simulink model "PIC_vector_concatenate_test"  (Simulink 6.6)
settings: Solver=FixedStepDiscrete  StartTime=0.0  StopTime=10.0  FixedStep=0.00001  RelTol=1e-3
libraries: dsPICdrivers x9, commutil2 x1, simulink x1
settings Model: Creator=Corey  LastModifiedBy=Corey  ProdHWDeviceType=16-bit Generic
settings OptimizationCC: OptimizeModelRefInitCode=on  LifeSpan=1
settings HardwareCC: ProdBitPerInt=16  ProdEndianess=LittleEndian  ProdWordSize=16  ProdHWDeviceType=16-bit Generic  TargetHWDeviceType=32-bit Generic
settings RTWCC: SystemTargetFile=dspic.tlc  TemplateMakefile=dspic_pic30_gcc.tmf  PostCodeGenCommand=dsPIC_Compile()  Description=Embedded Target for Microchip dsPIC (real-time)  ProcessScript=dspic_make_rtw_hook
settings CodeAppCC: IgnoreCustomStorageClasses=off
settings STFCustomTargetCC: TargetFcnLib=ansi_tfl_tmw.mat  GenFloatMathFcnCalls=ANSI_C  ModelReferenceCompliant=off  IncludeMdlTerminateFcn=off  CombineOutputUpdateFcns=on  SuppressErrorStatus=on  ERTCustomFileBanners=on  SupportContinuousTime=off  SupportNonInlinedSFcns=off  SystemTargetFile=dspic.tlc
settings ERTTargetCC: TargetFcnLib=ansi_tfl_tmw.mat  GenFloatMathFcnCalls=ANSI_C  ModelReferenceCompliant=off  IncludeMdlTerminateFcn=off  SuppressErrorStatus=on  ModelStepFunctionPrototypeControlCompliant=off  ExtModeMexFile=noextcomm  InlinedParameterPlacement=NonHierarchical  ERTSrcFileBannerTemplate=dsPIC_code_template.cgt  ERTHdrFileBannerTemplate=dsPIC_code_template.cgt  ERTDataSrcFileTemplate=dsPIC_code_template.cgt  ERTDataHdrFileTemplate=dsPIC_code_template.cgt  ERTCustomFileTemplate=dsPIC_main.tlc
settings CustomProperty: DataType=string  Value=J:\PROGRA~1\MATLAB\R2007a\rtw\bin\win32\gmake

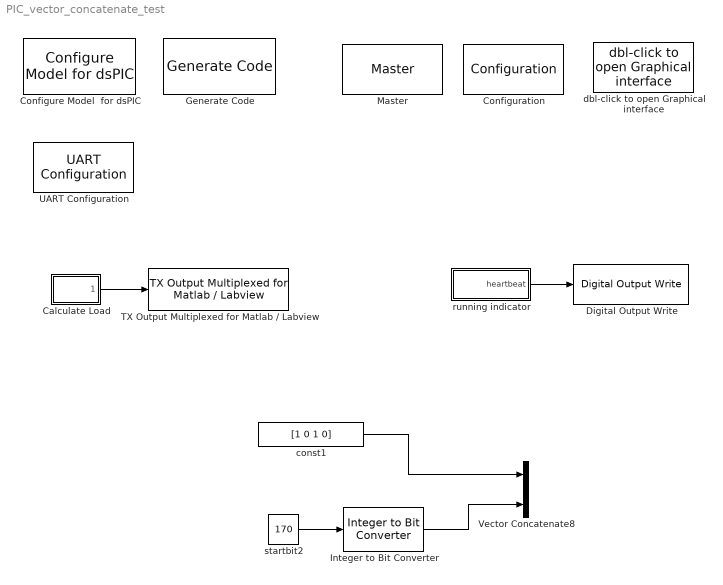
== system PIC_vector_concatenate_test ==
  Calculate Load : Subsystem
  Configuration : dsPICdrivers/Configuration  SystemSampleTime=-1  double64=off
  Configure Model  for dsPIC : dsPICdrivers/Simulink Configuration/Configure Model  for dsPIC
  Digital Output Write : dsPICdrivers/Digital I//O/Digital Output Write  Tag=dsPIC_Digital_Output  Priority=5  PORT=A  Pin=[0]  Simultaneous=off  OrderingInOutPopup=None
  Generate Code : dsPICdrivers/Simulink Configuration/Generate Code
  Integer to Bit Converter : commutil2/Integer to Bit Converter  nbits=8  outDtype=boolean
  Master : dsPICdrivers/Master  Tag=dsPIC_MASTER  Priority=1  TimeStepType=Timer1  picType=33fJ256GP710  fcy=40000000  Quartz_33f=8e6  PLLActive_33f=on  fcyDesired_33f=40000000  tmr1="[1  399  1.4211e-014]"  tmr1Info="Time Step : 1e-005  ;   Error : 1.4211e-014%  PR1=399"  tmr2345="[0  0  0  0  0  0  0  0]"  tmr2345cfg=[-1 -1 -1 -1 -1 -1 -1 -1]  IOautoConf=on  typePort="[ 10   0   0   0   0   0   0   0   0   0   0   0   0   0   0   0   0   0   0   0   0   0   0   0   0   0   0   0   0   0   0   0   0   0   0   0   0   0   0   0   0   0   0   0   0   0   0   0   0   0   0   0   0   0   0   0   0   0   0   0   0   0   0   0   0   0   0   0   0   0   0   0   0   0   0   0   0   0   0   0   0   0   0   0   4   5   0   0   0   0   0   0   0   0   0   0   0   0   0   0   0   0   0   0   0   0   0   0   0   0   0   0 ]"  TRIS="[ 65534  65535  65535  65535  65535  65535  65535 ]"  ADPCFG=0  MasterBusyPort=None  MasterOverloadPort=None  FOSC=Quartz (XT - HS)  ClockSwitchMonitor=Both disabled  TempProtection_33f=TEMP_ON  FPBOR=<empty>  PWRT=disable  MCLR=<empty>  PowerSave=off  OverrideFcy=off  NewFcy=1e6  PR2345="[65535  65535  65535  65535  65535  65535  65535  65535]"
  TX Output Multiplexed for Matlab / Labview : dsPICdrivers/Serial PORT/TX Output Multiplexed for Matlab // Labview  Tag=dsPIC_TX_Multiplexed  Priority=5  UART=2  CleverSpreadingChk=off  CleverSpreading=0  CHANNEL=[0]  CHANNELBLOCKED=[]  CHANNELBLOCKED_BITEWISE=0  Status=OK
  UART Configuration : dsPICdrivers/Serial PORT/UART Configuration  Tag=dsPIC_config_UART  Priority=2  UART=2  proposed_BAUD=115200  ALT_TX_RX=off  InterruptTxWhen=When Transmit Buffer is empty  TXInterruptPri=1  TxBufferSize=32  TXEN=on  InterruptRxWhen=When Receive Buffer is full (contain 4 characters)  RXInterruptPri=2  RxBufferSize=32  BAUD=115200  UxBRG=21  Info="UxBRG = 21   ||  Real Baud : 113636   ||  % error : -1.3573  ||  max 0.11364 Bytes / Step"  RealBaud=0
  Vector Concatenate8 : Concatenate  Mode=Vector
  const1 : Constant  Value=[1 0 1 0]  OutDataTypeMode=boolean  SampleTime=1/100
  dbl-click to open Graphical interface : dsPICdrivers/Serial PORT/dbl-click to open Graphical interface  SystemSampleTime=-1  Nothing=0
  running indicator : Subsystem
  startbit2 : Constant  Value=170  OutDataTypeMode=uint8  SampleTime=1/100
  wires:
  running indicator/1(heartbeat) -> Digital Output Write/1
  Calculate Load/1(% Load) -> TX Output Multiplexed for Matlab / Labview/1
  const1/1 -> Vector Concatenate8/1
  startbit2/1 -> Integer to Bit Converter/1
  Integer to Bit Converter/1 -> Vector Concatenate8/2

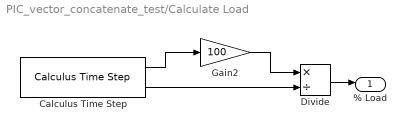
== system PIC_vector_concatenate_test/Calculate Load ==
  Calculus Time Step : dsPICdrivers/OTHERS/Calculus Time Step  Tag=dsPIC_CalculusTimeStep  SampleTime=0.01  PR1chk=on
  Divide : Product  Inputs=*/  OutDataTypeMode=uint16  OutScaling=2^-10
  Gain2 : Gain  Gain=100  OutDataTypeMode=Specify via dialog  OutDataType=uint(16)
  % Load : Outport
  wires:
  Calculus Time Step/2 -> Divide/2
  Calculus Time Step/1 -> Gain2/1
  Gain2/1 -> Divide/1
  Divide/1 -> % Load/1

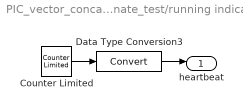
== system PIC_vector_concatenate_test/running indicator ==
  Counter Limited : simulink/Sources/Counter Limited  SystemSampleTime=-1  uplimit=1  tsamp=.5
  Data Type Conversion3 : DataTypeConversion  OutDataTypeMode=boolean
  heartbeat : Outport
  wires:
  Counter Limited/1 -> Data Type Conversion3/1
  Data Type Conversion3/1 -> heartbeat/1
